simulink model "solar_fopi_model2"  (R2024b)
settings: Solver=VariableStepAuto  StartTime=0.0  StopTime=1  RelTol=1e-3
libraries: spsIGBTDiodeLib x4, spsRMSLib x3, fod x2, simulink x2, spsCurrentMeasurementLib x1, spsDCVoltageSourceLib x1, spsSeriesRLCBranchLib x1, spsVoltageMeasurementLib x1, spspowerguiLib x1
settings Model: Creator=Beast23  LastModifiedBy=Uttam Kumar Thakur
settings SolverCC: ZeroCrossAlgorithm=Adaptive
settings DebuggingCC: IgnoredZcDiagnostic=none

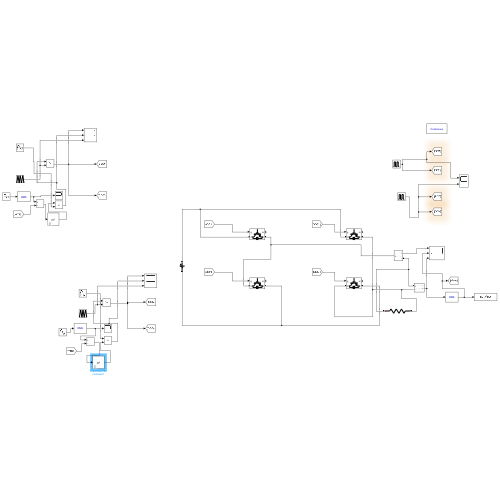
[thumbnail: Simulink's stored preview of the top-level diagram]
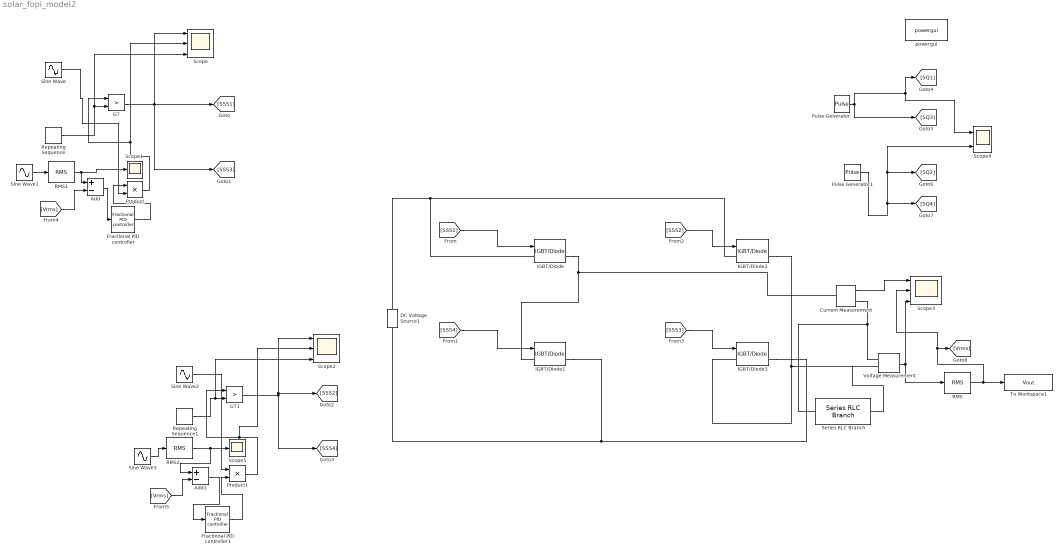
== system solar_fopi_model2 ==
  Add : Sum  Inputs=+-
  Add1 : Sum  Inputs=+-
  Current Measurement : spsCurrentMeasurementLib/Current Measurement  PhasorSimulation=off  OutputType=Complex  PSBequivalent=0
  DC Voltage Source1 : spsDCVoltageSourceLib/DC Voltage Source  Amplitude=200  Measurements=None
  Fractional PID controller : fod/Fractional PID controller  Kp=5  Ki=1  lambda=0.5  Kd=0  mic=0.5  freqRange=[0.01, 100]  N=10
      settings: SourceProductName=FOMCON Toolbox
  Fractional PID controller1 : fod/Fractional PID controller  Kp=5  Ki=1  lambda=0.5  Kd=0  mic=0.5  freqRange=[0.01, 100]  N=10
      settings: SourceProductName=FOMCON Toolbox
  GT : RelationalOperator  Operator=>  OutDataTypeStr=boolean  RndMeth=Simplest  InputSameDT=off
  GT1 : RelationalOperator  Operator=>  OutDataTypeStr=boolean  RndMeth=Simplest  InputSameDT=off
  IGBT/Diode{,1..3} (4 alike) : spsIGBTDiodeLib/IGBT//Diode  Ron=1e-3  Rs=1e5  Cs=inf  Measurements=on
  Product : Product
  Product1 : Product
  Pulse Generator : DiscretePulseGenerator  PulseType=Time based  Period=0.02  PulseWidth=50
  Pulse Generator1 : DiscretePulseGenerator  PulseType=Time based  Period=0.02  PulseWidth=50  PhaseDelay=0.01
  RMS : spsRMSLib/RMS  TrueRMS=on  Freq=50  RMSInit=120  Ts=0
  RMS1 : spsRMSLib/RMS  TrueRMS=on  Freq=50  RMSInit=120  Ts=0
  RMS2 : spsRMSLib/RMS  TrueRMS=on  Freq=50  RMSInit=120  Ts=0
  Repeating Sequence : simulink/Sources/Repeating Sequence  rep_seq_t=[0 0.02/40 0.02/20]  rep_seq_y=[0 2 0]
  Repeating Sequence1 : simulink/Sources/Repeating Sequence  rep_seq_t=[0 0.02/40 0.02/20]  rep_seq_y=[0 2 0]
  Scope : Scope  NumInputPorts=3
  Scope1 : Scope
  Scope2 : Scope  NumInputPorts=3
  Scope3 : Scope  NumInputPorts=3
  Scope4 : Scope  NumInputPorts=2
  Scope5 : Scope
  Series RLC Branch : spsSeriesRLCBranchLib/Series RLC Branch  LConnTagsString=__new0  RConnTagsString=__new0  BranchType=R  Resistance=0.1  Inductance=1e-3  SetiL0=off  InitialCurrent=0  Capacitance=1e-6  Setx0=off  InitialVoltage=0  Measurements=None
  Sine Wave : Sin  Frequency=2*pi*50  SampleTime=0
  Sine Wave1 : Sin  Amplitude=200  Frequency=2*pi*50  SampleTime=0
  Sine Wave2 : Sin  Frequency=2*pi*50  Phase=pi  SampleTime=0
  Sine Wave3 : Sin  Amplitude=200  Frequency=2*pi*50  Phase=pi  SampleTime=0
  To Workspace1 : ToWorkspace  VariableName=Vout  SaveFormat=Timeseries  SampleTime=-1
  Voltage Measurement : spsVoltageMeasurementLib/Voltage Measurement  PhasorSimulation=off  OutputType=Complex  PSBequivalent=0
  powergui : spspowerguiLib/powergui  Priority=1  SimulationMode=Continuous  SampleTime=50e-6  frequency=60  Iterations=50  frequencyindice=0  Pbase=100e6  ErrMax=1e-4  UnitsV=kV  UnitsW=MW  buscounter=0  FunctionMessages=off  echomessages=off  EnableUseOfTLC=off  CurrentSourceSwitches=off  DisableSnubberDevices=off  DisableRonSwitches=off  DisableVfSwitches=off  DisplayEquations=off  AutomaticDiscreteSolvers=off  SolverType=Tustin/Backward Euler (TBE)  Interpol=off  ExternalGateDelay=off  methode=off  Ts=100  x0status=blocks  SPID=on  SwTol=0  HookPort=off  NonlinearTolerance=1e-4  nMaxIteration=100  ContinueOnMaxIteration=off  RestoreLinks=warning  ResistiveCurrentMeasurement=off  Frange=[0:2:500]  Ylog=off  Xlog=on  ShowGrid=off  save=off  variable=ZData  structure=0  ZoomFFT=off  StartTime=0.0  cycles=1  DisplayStyle=1  fundamental=60  FreqAxis=off  MaxFrequency=1000  frequencyindicesteady=1  RmsSteady=1  display=off
  wires:
  GT/1 -> [SSS3], [SSS1], Scope/1
  Repeating Sequence/1 -> GT/2, Scope/3
  Sine Wave/1 -> Product/2
  Repeating Sequence1/1 -> Scope2/3, GT1/2
  GT1/1 -> [SSS4], Scope2/1, [SSS2]
  [SSS1] -> IGBT/Diode/1
  [SSS4] -> IGBT/Diode1/1
  [SSS3] -> IGBT/Diode3/1
  [SSS2] -> IGBT/Diode2/1
  Current Measurement/1 -> Scope3/1
  Voltage Measurement/1 -> RMS/1, Scope3/3
  Pulse Generator/1 -> [SQ3], [SQ1], Scope4/1
  Pulse Generator1/1 -> [SQ4], [SQ2], Scope4/2
  [Vrms] -> Add/2
  Product/1 -> GT/1, Scope/2
  [Vrms] -> Add1/2
  Sine Wave2/1 -> Product1/1
  Product1/1 -> Scope2/2, GT1/1
  RMS/1 -> To Workspace1/1, Scope3/2, [Vrms]
  Add/1 -> Fractional PID controller/1
  Fractional PID controller/1 -> Product/1
  Add1/1 -> Fractional PID controller1/1
  Fractional PID controller1/1 -> Product1/2
  RMS1/1 -> Add/1, Scope1/1
  Sine Wave1/1 -> RMS1/1
  RMS2/1 -> Add1/1, Scope5/1
  Sine Wave3/1 -> RMS2/1
  connections:
  IGBT/Diode/RConn1 -- Current Measurement/LConn1 -- IGBT/Diode1/LConn1
  IGBT/Diode2/RConn1 -- Series RLC Branch/RConn1 -- Voltage Measurement/LConn2 -- IGBT/Diode3/LConn1
  Current Measurement/RConn1 -- Series RLC Branch/LConn1 -- Voltage Measurement/LConn1
  IGBT/Diode3/RConn1 -- IGBT/Diode1/RConn1 -- DC Voltage Source1/LConn1
  IGBT/Diode2/LConn1 -- IGBT/Diode/LConn1 -- DC Voltage Source1/RConn1
